simulink model "arducopter"  (R2021a)
settings: Solver=FixedStepAuto  StartTime=0.0  StopTime=simIn.param.timeEnd  FixedStep=simIn.param.dt  RelTol=1e-3
undefined symbols (not defined in the file or in its folder): DiscIntNeverNeededParam, sim, simIn
libraries: simulink x35, slident x4, vrlib x1
(part 3 of 9)

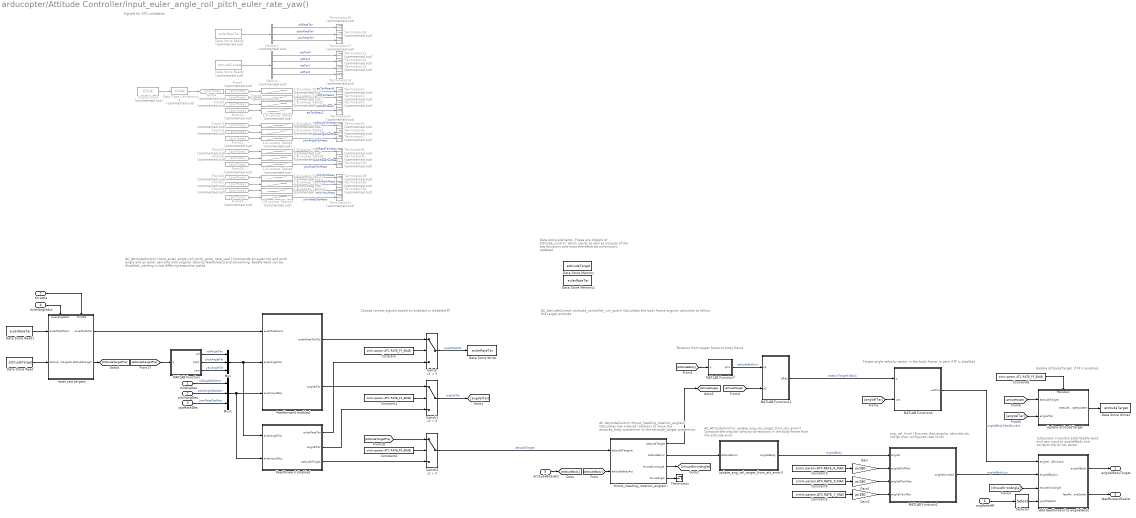
== system arducopter/Attitude Controller/input_euler_angle_roll_pitch_euler_rate_yaw() ==
  note: Signals for SITL validation
  note: Data store elements. These are objects of attitude_control, which inputs as well as outputs of the two functions and must therefore be continously updated
  note: Update attitudeTarget, if FF is enabled.
  note: Subsystem smoothly adds feedforward and yaw input to angVelBody and corrects the thrust vector
  note: Target angle velocity vector in the body frame. Is zero if FF is disabled
  note: Rotation from target frame to body frame
  note: Choose correct signals based on enabled or disabled FF
  note: AC_AttitudeControl::input_euler_angle_roll_pitch_euler_rate_yaw()
      | Commands an euler roll and pitch angle and an euler yaw arte with angular velocity feedforward and smoothing.
      | Feedforward can be disabled, yielding in two differing execution paths.
  note: AC_AttitudeControl::thrust_heading_rotation_angles()
      | Calculates two ordered rotations to move the attitude_body quaternion to the attitude_target quaternion.
  note: AC_AttitudeControl::update_ang_vel_target_from_att_error()
      | Compute the angular velocity corrections in the body frame from the attitude error.
  note: ang_vel_limit()
      | Ensures that angular velocites do not go over configured rate limits
  note: AC_AttitudeControl::attitude_controller_run_quat()
      | Calculates the body frame angular velocities to follow the target attitude
  rollAngDes : Inport
  pitchAngDes : Inport  Port=2
  yawRateDes : Inport  Port=3
  eulerAngleAct : Inport  Port=4
  attitudeBodyAct : Inport  Port=5
  angRatesBf : Inport  Port=6
  throttle : Inport  Port=7
  1-D Lookup Table : Lookup_n-D  Commented=on  NumberOfTableDimensions=1  BreakpointsForDimension1=simIn.signals.ATT.Time  Table=simIn.signals.ATT.attTarMeasW  InternalRulePriority=Speed  RndMeth=Simplest  InputSameDT=on
  1-D Lookup Table1 : Lookup_n-D  Commented=on  NumberOfTableDimensions=1  BreakpointsForDimension1=simIn.signals.ATT.Time  Table=simIn.signals.ATT.attTarMeasX  InternalRulePriority=Speed  RndMeth=Simplest  InputSameDT=on
  1-D Lookup Table10 : Lookup_n-D  Commented=on  NumberOfTableDimensions=1  BreakpointsForDimension1=simIn.signals.ATT.Time  Table=simIn.signals.ATT.CtrlRollIn  InternalRulePriority=Speed  RndMeth=Simplest  InputSameDT=on
  1-D Lookup Table11 : Lookup_n-D  Commented=on  NumberOfTableDimensions=1  BreakpointsForDimension1=simIn.signals.ATT.Time  Table=simIn.signals.ATT.CtrlPitchIn  InternalRulePriority=Speed  RndMeth=Simplest  InputSameDT=on
  1-D Lookup Table12 : Lookup_n-D  Commented=on  NumberOfTableDimensions=1  BreakpointsForDimension1=simIn.signals.ATT.Time  Table=simIn.signals.ATT.CtrlYawIn  InternalRulePriority=Speed  RndMeth=Simplest  InputSameDT=on
  1-D Lookup Table13 : Lookup_n-D  Commented=on  NumberOfTableDimensions=1  BreakpointsForDimension1=simIn.signals.ATT.Time  Table=simIn.signals.ATT.yawRateDesMeas  InternalRulePriority=Speed  RndMeth=Simplest  InputSameDT=on
  1-D Lookup Table2 : Lookup_n-D  Commented=on  NumberOfTableDimensions=1  BreakpointsForDimension1=simIn.signals.ATT.Time  Table=simIn.signals.ATT.attTarMeasY  InternalRulePriority=Speed  RndMeth=Simplest  InputSameDT=on
  1-D Lookup Table3 : Lookup_n-D  Commented=on  NumberOfTableDimensions=1  BreakpointsForDimension1=simIn.signals.ATT.Time  Table=simIn.signals.ATT.attTarMeasZ  InternalRulePriority=Speed  RndMeth=Simplest  InputSameDT=on
  1-D Lookup Table4 : Lookup_n-D  Commented=on  NumberOfTableDimensions=1  BreakpointsForDimension1=simIn.signals.ATT.Time  Table=simIn.signals.ATT.eulerAngTarMeasX  InternalRulePriority=Speed  RndMeth=Simplest  InputSameDT=on
  1-D Lookup Table5 : Lookup_n-D  Commented=on  NumberOfTableDimensions=1  BreakpointsForDimension1=simIn.signals.ATT.Time  Table=simIn.signals.ATT.eulerAngTarMeasY  InternalRulePriority=Speed  RndMeth=Simplest  InputSameDT=on
  1-D Lookup Table6 : Lookup_n-D  Commented=on  NumberOfTableDimensions=1  BreakpointsForDimension1=simIn.signals.ATT.Time  Table=simIn.signals.ATT.eulerAngTarMeasZ  InternalRulePriority=Speed  RndMeth=Simplest  InputSameDT=on
  1-D Lookup Table7 : Lookup_n-D  Commented=on  NumberOfTableDimensions=1  BreakpointsForDimension1=simIn.signals.ATT.Time  Table=simIn.signals.ATT.eulerRatTarMeasX  InternalRulePriority=Speed  RndMeth=Simplest  InputSameDT=on
  1-D Lookup Table8 : Lookup_n-D  Commented=on  NumberOfTableDimensions=1  BreakpointsForDimension1=simIn.signals.ATT.Time  Table=simIn.signals.ATT.eulerRatTarMeasY  InternalRulePriority=Speed  RndMeth=Simplest  InputSameDT=on
  1-D Lookup Table9 : Lookup_n-D  Commented=on  NumberOfTableDimensions=1  BreakpointsForDimension1=simIn.signals.ATT.Time  Table=simIn.signals.ATT.eulerRatTarMeasZ  InternalRulePriority=Speed  RndMeth=Simplest  InputSameDT=on
  Add feedforward to angVelBody : Subsystem
  Constant{,1..2,6} (4 alike) : Constant  Value=simIn.param.ATC.RATE_FF_ENAB
  Constant3 : Constant  Value=simIn.param.ATC.RATE_R_MAX
  Constant4 : Constant  Value=simIn.param.ATC.RATE_P_MAX
  Constant5 : Constant  Value=simIn.param.ATC.RATE_Y_MAX
  Data Store Memory : DataStoreMemory  DataStoreName=attitudeTarget  ReadBeforeWriteMsg=warning  WriteAfterWriteMsg=warning  WriteAfterReadMsg=warning  InitialValue=simIn.init.ATT.attitudeTarget  ShowAdditionalParam=off  OutDataTypeStr=single
  Data Store Memory1 : DataStoreMemory  DataStoreName=eulerRateTar  ReadBeforeWriteMsg=warning  WriteAfterWriteMsg=warning  WriteAfterReadMsg=warning  InitialValue=simIn.init.ATT.eulerRateTar  ShowAdditionalParam=off  OutDataTypeStr=single
  Data Store Read : DataStoreRead  DataStoreName=attitudeTarget  IndexOptions=Index vector (dialog)  Indices=1  OutputSizes=1
  Data Store Read1 : DataStoreRead  DataStoreName=eulerRateTar  IndexOptions=Index vector (dialog)  Indices=1  OutputSizes=1
  Data Store Read3 : DataStoreRead  Commented=on  DataStoreName=attitudeTarget  IndexOptions=Index vector (dialog)  Indices=1  OutputSizes=1
  Data Store Read4 : DataStoreRead  Commented=on  DataStoreName=eulerRateTar  IndexOptions=Index vector (dialog)  Indices=1  OutputSizes=1
  Data Store Write : DataStoreWrite  DataStoreName=eulerRateTar  IndexOptions=Index vector (dialog)  Indices=1  OutputSizes=1
  Data Store Write1 : DataStoreWrite  DataStoreName=attitudeTarget  IndexOptions=Index vector (dialog)  Indices=1  OutputSizes=1
  Data Type Conversion4 : DataTypeConversion  Commented=on  OutDataTypeStr=single
  Demux : Demux  Commented=on
  Demux1 : Demux  Commented=on  Outputs=3
  Digital Clock : DigitalClock  Commented=on  SampleTime=sim.param.dt
  Feedforward disabled : Subsystem
  Feedforward enabled : Subsystem
  From{7..16,19..22} (14 alike) : From  Commented=on  GotoTag=simTime
  Gain : Gain  Gain=pi/180
  Gain1 : Gain  Gain=pi/180
  Gain2 : Gain  Gain=pi/180
  Goto4 : Goto  Commented=on  GotoTag=simTime
  MATLAB Function : MATLAB Function  TreatAsAtomicUnit=on
  MATLAB Function11 : MATLAB Function  TreatAsAtomicUnit=on
  MATLAB Function2 : MATLAB Function  TreatAsAtomicUnit=on
  MATLAB Function4 : MATLAB Function  TreatAsAtomicUnit=on
  MATLAB Function7 : MATLAB Function  TreatAsAtomicUnit=on
  Mux : Mux  Inputs=3
  Mux1 : Mux  Inputs=3
  Selector : Selector  InputPortWidth=3  IndexOptions=Index vector (dialog)  Indices=[3]  OutputSizes=1
  Switch : Switch  Criteria=u2 > Threshold
  Switch1 : Switch  Criteria=u2 > Threshold
  Switch2 : Switch  Criteria=u2 > Threshold
  Terminator : Terminator
  Terminator{1..21} (21 alike) : Terminator  Commented=on
  Update attitudeTarget : Subsystem
      settings: PortSchema="{\"entries\":[{\"content\":{\"sides\":[{\"content\":{\"connectorIds\":[\"In1\",\"In2\"]},\"type\":\"ConnectorPlacement.EquallySpacedRectSide\",\"uuid\":\"677f2474-a933-4351-a18c-d191f7c74006\"},{\"content\":{\"connectorIds\":[\"Out1\"],\"side\":\"RIGHT\"},\"type\":\"ConnectorPlacement.EquallySpacedRectSide\",\"uuid\":\"e9b9097f-3644-4a9a-8149-04c97bd90a0c\"},{\"content\":{\"connectorIds\":[\"In3\"],\"side\":\"TOP\"},\"type\":\"ConnectorPlacement.EquallySpacedRectSide\",\"uuid\":\"2b4d5a13-4fc6-40d8-be4c-f1f4571d6c96\"}]},\"type\":\"ConnectorPlacement.EquallySpacedConnector\",\"uuid\":\"62980eaf-3b78-41ff-aa7a-c4a8a9508ced\"}],\"packageUris\":[\"http://schema.mathworks.com/mf0/Connector/R2020b\"],\"version\":\"1.0\"}"
  reset yaw targets : Subsystem
      settings: PortSchema="{\"entries\":[{\"content\":{\"sides\":[{\"content\":{\"connectorIds\":[\"In1\",\"In2\"]},\"type\":\"ConnectorPlacement.EquallySpacedRectSide\",\"uuid\":\"29284c76-4388-4ab2-b640-2aa249641a5e\"},{\"content\":{\"connectorIds\":[\"Out1\",\"Out2\"],\"side\":\"RIGHT\"},\"type\":\"ConnectorPlacement.EquallySpacedRectSide\",\"uuid\":\"b3687b33-33ad-4cf1-ba70-eea9295fb5e4\"},{\"content\":{\"connectorIds\":[\"In3\",\"In4\"],\"side\":\"TOP\"},\"type\":\"ConnectorPlacement.EquallySpacedRectSide\",\"uuid\":\"b547cb73-472d-403b-8f7c-c78a9fbe5228\"}]},\"type\":\"ConnectorPlacement.EquallySpacedConnector\",\"uuid\":\"31dffed6-fd3b-4288-90b3-a2b7b520dc2f\"}],\"packageUris\":[\"http://schema.mathworks.com/mf0/Connector/R2020b\"],\"version\":\"1.0\"}"
  thrust_heading_rotation_angles() : Subsystem
  update_ang_vel_target_from_att_error() : Subsystem
  angVelBodyTarget : Outport
  feedforwardScaler : Outport  Port=2
  wires:
  MATLAB Function/3(yaw) -> Mux/3  "yawAngleTar"
  MATLAB Function/2(pitch) -> Mux/2  "pitchAngleTar"
  MATLAB Function/1(roll) -> Mux/1  "rollAngleTar"
  Mux/1 -> Feedforward disabled/1(eulerAngleTar), Feedforward enabled/2(eulerAngleTar)
  rollAngDes/1 -> Mux1/1  "rollAngleDesNew"
  pitchAngDes/1 -> Mux1/2  "pitchAngleDesNew"
  yawRateDes/1 -> Mux1/3  "yawRateDesNew"
  Mux1/1 -> Feedforward enabled/3(eulerInputDes), Feedforward disabled/2(eulerInputDes)
  Data Store Read1/1 -> reset yaw targets/1(eulerRateTarIn)
  Feedforward enabled/1(eulerRateTarOut) -> Switch/1
  Feedforward disabled/1(eulerRateTar) -> Switch/3
  Feedforward enabled/2(angVelTar) -> Switch1/1
  Constant/1 -> Switch/2
  Feedforward disabled/2(angVelTar) -> Switch1/3
  Switch/1 -> Data Store Write/1  "eulerRateTar"
  Switch1/1 -> [angVelTar]  "angVelTar"
  Constant1/1 -> Switch1/2
  Constant2/1 -> Switch2/2
  [attitudeTargetPre] -> Switch2/1
  Feedforward disabled/3(attitudeTarget) -> Switch2/3
  Switch2/1 -> thrust_heading_rotation_angles()/1(attitudeTargetIn)  "attitudeTarget"
  [attitudeBody] -> thrust_heading_rotation_angles()/2(attitudeBodyAct)
  thrust_heading_rotation_angles()/4(thrustAngle) -> Terminator/1
  thrust_heading_rotation_angles()/2(attitudeError) -> update_ang_vel_target_from_att_error()/1(attitudeError)
  Constant4/1 -> Gain1/1
  Constant3/1 -> Gain/1
  Gain2/1 -> MATLAB Function2/4(angVelYawMax)
  Gain1/1 -> MATLAB Function2/3(angVelPitchMax)
  Constant5/1 -> Gain2/1
  Gain/1 -> MATLAB Function2/2(angVelRollMax)
  update_ang_vel_target_from_att_error()/1(angVelBody) -> MATLAB Function2/1(angVel)  "angVelBody"
  attitudeBodyAct/1 -> [attitudeBody]
  thrust_heading_rotation_angles()/1(attitudeTarget) -> [attitudeTarget]
  [attitudeBody] -> MATLAB Function7/1(q)
  MATLAB Function7/1(qInv) -> MATLAB Function11/1(q1)  "attitudeBodyInv"
  MATLAB Function11/1(qRes) -> MATLAB Function4/1(q)  "rotationTargetToBody"
  [angVelTar] -> MATLAB Function4/2(vec)
  MATLAB Function4/1(vecRot) -> Add feedforward to angVelBody/1(angVelBodyFeedforward)  "angVelBodyFeedforward"
  thrust_heading_rotation_angles()/3(thrustErrorAngle) -> [thrustErrorAngle]
  MATLAB Function2/1(angVelLimited) -> Add feedforward to angVelBody/2(angVelBodyIn)  "angVelBodyLim"
  [thrustErrorAngle] -> Add feedforward to angVelBody/3(thurstErrorAngle)
  angRatesBf/1 -> Selector/1
  Selector/1 -> Add feedforward to angVelBody/4(yawRateAct)
  [attitudeTarget] -> MATLAB Function11/2(q2)
  [angVelTar] -> Update attitudeTarget/2(angVelTar)
  Add feedforward to angVelBody/1(angVelBody) -> angVelBodyTarget/1
  [attitudeTarget] -> Update attitudeTarget/1(attitudeTarget)
  Update attitudeTarget/1(attitudeTargetUpdate) -> Data Store Write1/1
  Constant6/1 -> Update attitudeTarget/3(ffEnabled)
  Add feedforward to angVelBody/2(feedforwardScaler) -> feedforwardScaler/1
  Data Type Conversion4/1 -> Goto4/1
  Digital Clock/1 -> Data Type Conversion4/1
  From7/1 -> 1-D Lookup Table/1
  From8/1 -> 1-D Lookup Table1/1
  From9/1 -> 1-D Lookup Table2/1
  From10/1 -> 1-D Lookup Table3/1
  From11/1 -> 1-D Lookup Table6/1
  From13/1 -> 1-D Lookup Table5/1
  From12/1 -> 1-D Lookup Table4/1
  From15/1 -> 1-D Lookup Table7/1
  From16/1 -> 1-D Lookup Table8/1
  From14/1 -> 1-D Lookup Table9/1
  1-D Lookup Table/1 -> Terminator1/1  "attTarMeasW"
  1-D Lookup Table1/1 -> Terminator2/1  "attTarMeasX"
  1-D Lookup Table2/1 -> Terminator3/1  "attTarMeasY"
  1-D Lookup Table3/1 -> Terminator4/1  "attTarMeasZ"
  1-D Lookup Table6/1 -> Terminator7/1  "yawAngleTarMeas"
  1-D Lookup Table5/1 -> Terminator6/1  "pitchAngleTarMeas"
  1-D Lookup Table4/1 -> Terminator5/1  "rollAngleTarMeas"
  1-D Lookup Table7/1 -> Terminator8/1  "rollRateTarMeas"
  1-D Lookup Table8/1 -> Terminator9/1  "pitchRateTarMeas"
  1-D Lookup Table9/1 -> Terminator10/1  "yawRateTarMeas"
  Data Store Read3/1 -> Demux/1
  Demux/4 -> Terminator14/1  "attTarZ"
  Demux/3 -> Terminator13/1  "attTarY"
  Demux/2 -> Terminator12/1  "attTarX"
  Demux/1 -> Terminator11/1  "attTarW"
  Data Store Read4/1 -> Demux1/1
  Demux1/1 -> Terminator15/1  "rollRateTar"
  Demux1/2 -> Terminator16/1  "pitchRateTar"
  Demux1/3 -> Terminator17/1  "yawRateTar"
  Data Store Read/1 -> reset yaw targets/2(attitudeTargetIn)
  reset yaw targets/1(eulerRateTar) -> Feedforward enabled/1(eulerRateTarIn)
  eulerAngleAct/1 -> reset yaw targets/3(eulerAngleAct)
  [attitudeTargetPre] -> MATLAB Function/1(q)
  reset yaw targets/2(attitudeTarget) -> [attitudeTargetPre]
  throttle/1 -> reset yaw targets/4(throttle)
  From19/1 -> 1-D Lookup Table12/1
  From21/1 -> 1-D Lookup Table11/1
  From20/1 -> 1-D Lookup Table10/1
  From22/1 -> 1-D Lookup Table13/1
  1-D Lookup Table10/1 -> Terminator19/1  "ctrlInRollMeas"
  1-D Lookup Table11/1 -> Terminator20/1  "ctrlInPitchMeas"
  1-D Lookup Table12/1 -> Terminator18/1  "ctrlInYawMeas"
  1-D Lookup Table13/1 -> Terminator21/1  "yawRateDesMeas"

== system arducopter/Lowpass2p/Lowpass Pitch ==
  u : Inport
  sampleFreq : Inport  Port=2
  cutoffFreq : Inport  Port=3
  Data Store Memory1 : DataStoreMemory  DataStoreName=delElem2  ReadBeforeWriteMsg=warning  WriteAfterWriteMsg=warning  WriteAfterReadMsg=warning  ShowAdditionalParam=off  OutDataTypeStr=single
  Data Store Memory10 : DataStoreMemory  DataStoreName=delElem1  ReadBeforeWriteMsg=warning  WriteAfterWriteMsg=warning  WriteAfterReadMsg=warning  ShowAdditionalParam=off  OutDataTypeStr=single
  Lowpass2p : MATLAB Function  TreatAsAtomicUnit=on
  y : Outport
  wires:
  u/1 -> Lowpass2p/1(u)
  cutoffFreq/1 -> Lowpass2p/3(cutoffFreq)
  sampleFreq/1 -> Lowpass2p/2(sampleFreq)
  Lowpass2p/1(y) -> y/1

== system arducopter/Lowpass2p/Lowpass Roll ==
  u : Inport
  sampleFreq : Inport  Port=2
  cutoffFreq : Inport  Port=3
  Data Store Memory1 : DataStoreMemory  DataStoreName=delElem2  ReadBeforeWriteMsg=warning  WriteAfterWriteMsg=warning  WriteAfterReadMsg=warning  ShowAdditionalParam=off  OutDataTypeStr=single
  Data Store Memory10 : DataStoreMemory  DataStoreName=delElem1  ReadBeforeWriteMsg=warning  WriteAfterWriteMsg=warning  WriteAfterReadMsg=warning  ShowAdditionalParam=off  OutDataTypeStr=single
  Lowpass2p : MATLAB Function  TreatAsAtomicUnit=on
  y : Outport
  wires:
  Lowpass2p/1(y) -> y/1
  sampleFreq/1 -> Lowpass2p/2(sampleFreq)
  cutoffFreq/1 -> Lowpass2p/3(cutoffFreq)
  u/1 -> Lowpass2p/1(u)

== system arducopter/Lowpass2p/Lowpass Yaw ==
  u : Inport
  sampleFreq : Inport  Port=2
  cutoffFreq : Inport  Port=3
  Data Store Memory1 : DataStoreMemory  DataStoreName=delElem2  ReadBeforeWriteMsg=warning  WriteAfterWriteMsg=warning  WriteAfterReadMsg=warning  ShowAdditionalParam=off  OutDataTypeStr=single
  Data Store Memory10 : DataStoreMemory  DataStoreName=delElem1  ReadBeforeWriteMsg=warning  WriteAfterWriteMsg=warning  WriteAfterReadMsg=warning  ShowAdditionalParam=off  OutDataTypeStr=single
  Lowpass2p : MATLAB Function  TreatAsAtomicUnit=on
  y : Outport
  wires:
  u/1 -> Lowpass2p/1(u)
  cutoffFreq/1 -> Lowpass2p/3(cutoffFreq)
  sampleFreq/1 -> Lowpass2p/2(sampleFreq)
  Lowpass2p/1(y) -> y/1

== system arducopter/Position Controller/P Position z ==
  note: AC_PosControl::update_z_controller() - Position controller
  note: Feed-Forward component
      | update_z_controller()
  note: AC_P_1D::update_all()
      | These two Matlab functions represent the update_all() function of the AC_P_1D class. The function basically consists of two parts, the error
      | calculation with limiting (implemented by calc_err) and the square root controller (implemented by sqrt_controller).
  note: Testrun inputs
  note: Parameter
  note: AC_PosControl::set_correction_speed_accel_z()
  posTar : Inport
  posAct : Inport  Port=2
  velDes : Inport  Port=3
  Calculate error : MATLAB Function  TreatAsAtomicUnit=on
  Constant : Constant  Value=0  OutDataTypeStr=single
  Data Type Conversion : DataTypeConversion  OutDataTypeStr=single
  IC1 : InitialCondition  Value=simIn.init.PIDA.posTar
  Product : Product
  Scale Factor Z : Subsystem
  Set vertical speed & acceleration limit : Subsystem
  Square Root Controller : MATLAB Function  TreatAsAtomicUnit=on
  Sum : Sum  Inputs=++|
  dt : Constant  Value=simIn.param.dt
  ekf_type : Constant  Value=simIn.param.EKF_TYPE
  kp_pos : Constant  Value=simIn.param.PSCD.P_POS
  speedDnMax : Constant  Value=simIn.param.PSCD.VEL_MAX_DN
  speedUpMax : Constant  Value=simIn.param.PSCD.VEL_MAX_UP
  zAccMax : Constant  Value=simIn.param.PSCD.ACC_MAX_Z
  velTar : Outport
  posTarUpd : Outport  Port=2
  posErr : Outport  Port=3
  wires:
  speedDnMax/1 -> [dnSpeedMax]
  posAct/1 -> Calculate error/2(act)
  posTar/1 -> IC1/1
  speedUpMax/1 -> [upSpeedMax]
  zAccMax/1 -> [zAccMax]
  kp_pos/1 -> [kpPos]
  [errMin] -> Calculate error/3(err_min)
  [errMax] -> Calculate error/4(err_max)
  [dnSpeedMax] -> Set vertical speed & acceleration limit/1(outMin)
  [upSpeedMax] -> Set vertical speed & acceleration limit/2(outMax)
  [zAccMax] -> Set vertical speed & acceleration limit/3(DoutMax)
  Constant/1 -> Set vertical speed & acceleration limit/4(D2OutMax)
  Set vertical speed & acceleration limit/1(errMin) -> [errMin]
  Set vertical speed & acceleration limit/2(errMax) -> [errMax]
  [error] -> Square Root Controller/1(err)
  Set vertical speed & acceleration limit/3(D1max) -> [D1max]
  [D1max] -> Square Root Controller/3(second_ord_lim)
  [kpPos] -> Square Root Controller/2(p)
  dt/1 -> Data Type Conversion/1
  [dt] -> Square Root Controller/4(dt)
  ekf_type/1 -> [ekfType]
  [ekfType] -> Scale Factor Z/1(ekfType)
  Square Root Controller/1(correction_rate) -> Product/2
  Scale Factor Z/1(scale_z) -> Product/1
  Calculate error/1(tar_new) -> posTarUpd/1
  Product/1 -> Sum/2
  velDes/1 -> Sum/1
  Sum/1 -> velTar/1
  Data Type Conversion/1 -> [dt]
  IC1/1 -> Calculate error/1(tar)
  Calculate error/2(err) -> [error]
  [error] -> posErr/1
  [kpPos] -> Set vertical speed & acceleration limit/5(kp)

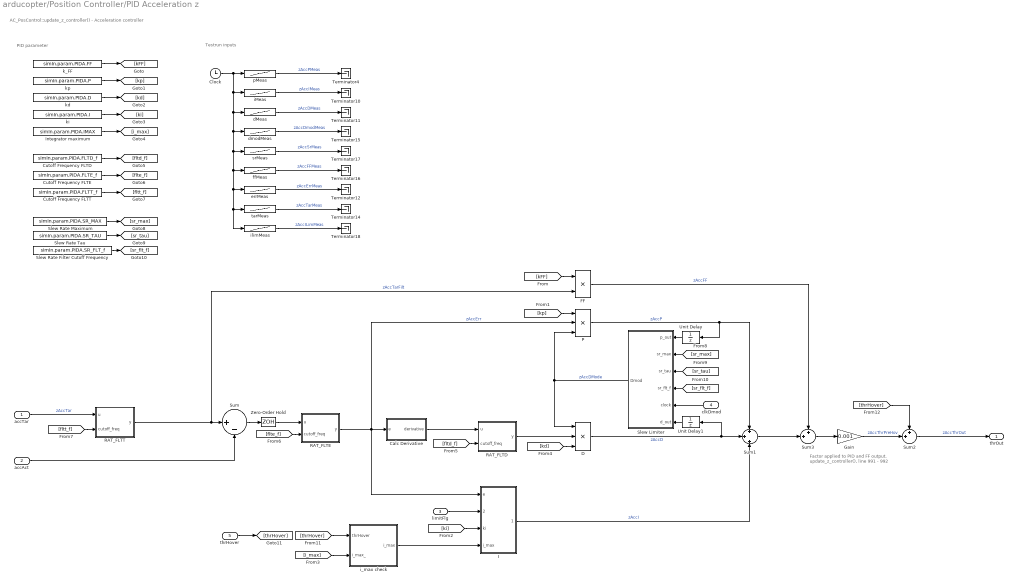
== system arducopter/Position Controller/PID Acceleration z ==
  note: Factor applied to PID and FF output.
      | update_z_controller(), line 991 - 992
  note: AC_PosControl::update_z_controller() - Acceleration controller
  note: PID parameter
  note: Testrun inputs
  accTar : Inport
  accAct : Inport  Port=2
  limitFlg : Inport  Port=3
  clkDmod : Inport  Port=4
  thrHover : Inport  Port=5
  Calc Derivative : Subsystem
  Clock : Clock
  Cutoff Frequency FLTD : Constant  Value=simIn.param.PIDA.FLTD_f
  Cutoff Frequency FLTE : Constant  Value=simIn.param.PIDA.FLTE_f
  Cutoff Frequency FLTT : Constant  Value=simIn.param.PIDA.FLTT_f
  D : Product  Inputs=3
  FF : Product
  Gain : Gain  Gain=0.001
  I : Subsystem
  Integrator maximum : Constant  Value=simIn.param.PIDA.IMAX
  P : Product  Inputs=3
  RAT_FLTD : Subsystem  TreatAsAtomicUnit=on  SystemSampleTime=simIn.param.dt
  RAT_FLTE : Subsystem  TreatAsAtomicUnit=on  SystemSampleTime=simIn.param.dt
  RAT_FLTT : Subsystem  TreatAsAtomicUnit=on  SystemSampleTime=simIn.param.dt
  Slew Limiter : Subsystem
  Slew Rate Filter Cutoff Frequency : Constant  Value=simIn.param.PIDA.SR_FLT_f
  Slew Rate Maximum : Constant  Value=simIn.param.PIDA.SR_MAX
  Slew Rate Tau : Constant  Value=simIn.param.PIDA.SR_TAU
  Sum : Sum  Inputs=|+-
  Sum1 : Sum  Inputs=+|+|+
  Sum2 : Sum  Inputs=++|  OutDataTypeStr=single
  Sum3 : Sum  Inputs=++|  OutDataTypeStr=single
  Terminator{4,10..12,14..18} (9 alike) : Terminator
  Unit Delay : UnitDelay  InitialCondition=simIn.init.PIDA.P  SampleTime=-1  HasFrameUpgradeWarning=on
  Unit Delay1 : UnitDelay  InitialCondition=simIn.init.PIDA.D  SampleTime=-1  HasFrameUpgradeWarning=on
  Zero-Order Hold : ZeroOrderHold  SampleTime=-1
  dMeas : Lookup_n-D  NumberOfTableDimensions=1  BreakpointsForDimension1=simIn.signals.PIDR.Time  Table=simIn.signals.PIDR.D  InternalRulePriority=Speed  RndMeth=Simplest  InputSameDT=on
  dmodMeas : Lookup_n-D  NumberOfTableDimensions=1  BreakpointsForDimension1=simIn.signals.PIDA.Time  Table=simIn.signals.PIDA.DMod  InternalRulePriority=Speed  RndMeth=Simplest  InputSameDT=on
  errMeas : Lookup_n-D  NumberOfTableDimensions=1  BreakpointsForDimension1=simIn.signals.PIDA.Time  Table=simIn.signals.PIDA.Err  InternalRulePriority=Speed  RndMeth=Simplest  InputSameDT=on
  ffMeas : Lookup_n-D  NumberOfTableDimensions=1  BreakpointsForDimension1=simIn.signals.PIDA.Time  Table=simIn.signals.PIDA.FF  InternalRulePriority=Speed  RndMeth=Simplest  InputSameDT=on
  iMeas : Lookup_n-D  NumberOfTableDimensions=1  BreakpointsForDimension1=simIn.signals.PIDA.Time  Table=simIn.signals.PIDA.I  InternalRulePriority=Speed  RndMeth=Simplest  InputSameDT=on
  i_max check : Subsystem
  ilimMeas : Lookup_n-D  NumberOfTableDimensions=1  BreakpointsForDimension1=simIn.signals.PIDA.Time  Table=simIn.signals.PIDA.ILimit  InternalRulePriority=Speed  RndMeth=Simplest  InputSameDT=on
  k_FF : Constant  Value=simIn.param.PIDA.FF
  kd : Constant  Value=simIn.param.PIDA.D
  ki : Constant  Value=simIn.param.PIDA.I
  kp : Constant  Value=simIn.param.PIDA.P
  pMeas : Lookup_n-D  NumberOfTableDimensions=1  BreakpointsForDimension1=simIn.signals.PIDA.Time  Table=simIn.signals.PIDA.P  InternalRulePriority=Speed  RndMeth=Simplest  InputSameDT=on
  srMeas : Lookup_n-D  NumberOfTableDimensions=1  BreakpointsForDimension1=simIn.signals.PIDA.Time  Table=simIn.signals.PIDA.SRate  InternalRulePriority=Speed  RndMeth=Simplest  InputSameDT=on
  tarMeas : Lookup_n-D  NumberOfTableDimensions=1  BreakpointsForDimension1=simIn.signals.PSCD.Time  Table=simIn.signals.PSCD.zAccTar  InternalRulePriority=Speed  RndMeth=Simplest  InputSameDT=on
  thrOut : Outport
  wires:
  RAT_FLTD/1(y) -> D/2
  Sum1/1 -> Sum3/2
  limitFlg/1 -> I/2(limitFlg)
  P/1 -> Unit Delay/1, Sum1/1  "zAccP"
  Calc Derivative/1(derivative) -> RAT_FLTD/1(u)
  Sum/1 -> Zero-Order Hold/1
  D/1 -> Unit Delay1/1, Sum1/2  "zAccD"
  I/1(integrator) -> Sum1/3  "zAccI"
  FF/1 -> Sum3/1  "zAccFF"
  Sum3/1 -> Gain/1
  RAT_FLTT/1(y) -> FF/2, Sum/1  "zAccTarFilt"
  Zero-Order Hold/1 -> RAT_FLTE/1(u)
  k_FF/1 -> [kFF]
  kp/1 -> [kp]
  kd/1 -> [kd]
  ki/1 -> [ki]
  Integrator maximum/1 -> [i_max]
  Cutoff Frequency FLTD/1 -> [fltd_f]
  Cutoff Frequency FLTE/1 -> [flte_f]
  Cutoff Frequency FLTT/1 -> [fltt_f]
  [kFF] -> FF/1
  [kp] -> P/1
  [ki] -> I/3(ki)
  [kd] -> D/3
  [fltd_f] -> RAT_FLTD/2(cutoff_freq)
  [flte_f] -> RAT_FLTE/2(cutoff_freq)
  [fltt_f] -> RAT_FLTT/2(cutoff_freq)
  RAT_FLTE/1(y) -> P/2, Calc Derivative/1(e), I/1(e)  "zAccErr"
  Slew Rate Filter Cutoff Frequency/1 -> [sr_flt_f]
  Slew Rate Maximum/1 -> [sr_max]
  Slew Rate Tau/1 -> [sr_tau]
  Slew Limiter/1(Dmod) -> D/1, P/3  "zAccDMode"
  Unit Delay/1 -> Slew Limiter/1(p_out)
  Unit Delay1/1 -> Slew Limiter/6(d_out)
  [sr_max] -> Slew Limiter/2(sr_max)
  [sr_tau] -> Slew Limiter/3(sr_tau)
  [sr_flt_f] -> Slew Limiter/4(sr_flt_f)
  clkDmod/1 -> Slew Limiter/5(clock)
  [thrHover] -> i_max check/1(thrHover)
  [i_max] -> i_max check/2(i_max_)
  i_max check/1(i_max) -> I/4(i_max)
  Sum2/1 -> thrOut/1  "zAccThrOut"
  thrHover/1 -> [thrHover]
  Gain/1 -> Sum2/2  "zAccThrPreHov"
  [thrHover] -> Sum2/1
  Clock/1 -> ilimMeas/1, tarMeas/1, errMeas/1, ffMeas/1, srMeas/1, dmodMeas/1, dMeas/1, iMeas/1, pMeas/1
  dmodMeas/1 -> Terminator15/1  "zAccDmodMeas"
  ilimMeas/1 -> Terminator18/1  "zAccILimMeas"
  srMeas/1 -> Terminator17/1  "zAccSrMeas"
  iMeas/1 -> Terminator10/1  "zAccIMeas"
  ffMeas/1 -> Terminator16/1  "zAccFFMeas"
  pMeas/1 -> Terminator4/1  "zAccPMeas"
  errMeas/1 -> Terminator12/1  "zAccErrMeas"
  tarMeas/1 -> Terminator14/1  "zAccTarMeas"
  dMeas/1 -> Terminator11/1  "zAccDMeas"
  accAct/1 -> Sum/2
  accTar/1 -> RAT_FLTT/1(u)  "zAccTar"

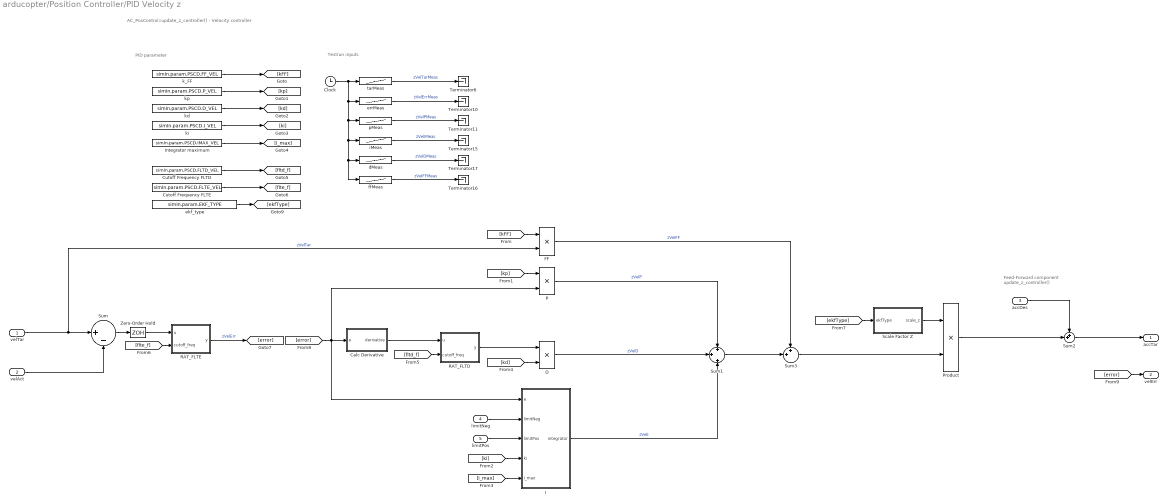
== system arducopter/Position Controller/PID Velocity z ==
  note: PID parameter
  note: Testrun inputs
  note: Feed-Forward component
      | update_z_controller()
  note: AC_PosControl::update_z_controller() - Velocity controller
  velTar : Inport
  velAct : Inport  Port=2
  accDes : Inport  Port=3
  limitNeg : Inport  Port=4
  limitPos : Inport  Port=5
  Calc Derivative : Subsystem
  Clock : Clock
  Cutoff Frequency FLTD : Constant  Value=simIn.param.PSCD.FLTD_VEL
  Cutoff Frequency FLTE : Constant  Value=simIn.param.PSCD.FLTE_VEL
  D : Product
  FF : Product
  I : Subsystem
  Integrator maximum : Constant  Value=simIn.param.PSCD.IMAX_VEL
  P : Product
  Product : Product
  RAT_FLTD : Subsystem  TreatAsAtomicUnit=on  SystemSampleTime=simIn.param.dt
  RAT_FLTE : Subsystem  TreatAsAtomicUnit=on  SystemSampleTime=simIn.param.dt
  Scale Factor Z : Subsystem
  Sum : Sum  Inputs=|+-
  Sum1 : Sum  Inputs=+|+|+
  Sum2 : Sum  Inputs=++|
  Sum3 : Sum  Inputs=++|  OutDataTypeStr=single
  Terminator{6,10..11,15..17} (6 alike) : Terminator
  Zero-Order Hold : ZeroOrderHold  SampleTime=-1
  dMeas : Lookup_n-D  NumberOfTableDimensions=1  BreakpointsForDimension1=simIn.signals.PCVZ.Time  Table=simIn.signals.PCVZ.D  InternalRulePriority=Speed  RndMeth=Simplest  InputSameDT=on
  ekf_type : Constant  Value=simIn.param.EKF_TYPE
  errMeas : Lookup_n-D  NumberOfTableDimensions=1  BreakpointsForDimension1=simIn.signals.PCVZ.Time  Table=simIn.signals.PCVZ.Err  InternalRulePriority=Speed  RndMeth=Simplest  InputSameDT=on
  ffMeas : Lookup_n-D  NumberOfTableDimensions=1  BreakpointsForDimension1=simIn.signals.PCVZ.Time  Table=simIn.signals.PCVZ.FF  InternalRulePriority=Speed  RndMeth=Simplest  InputSameDT=on
  iMeas : Lookup_n-D  NumberOfTableDimensions=1  BreakpointsForDimension1=simIn.signals.PCVZ.Time  Table=simIn.signals.PCVZ.I  InternalRulePriority=Speed  RndMeth=Simplest  InputSameDT=on
  k_FF : Constant  Value=simIn.param.PSCD.FF_VEL
  kd : Constant  Value=simIn.param.PSCD.D_VEL
  ki : Constant  Value=simIn.param.PSCD.I_VEL
  kp : Constant  Value=simIn.param.PSCD.P_VEL
  pMeas : Lookup_n-D  NumberOfTableDimensions=1  BreakpointsForDimension1=simIn.signals.PCVZ.Time  Table=simIn.signals.PCVZ.P  InternalRulePriority=Speed  RndMeth=Simplest  InputSameDT=on
  tarMeas : Lookup_n-D  NumberOfTableDimensions=1  BreakpointsForDimension1=simIn.signals.PSCD.Time  Table=simIn.signals.PSCD.zVelTar  InternalRulePriority=Speed  RndMeth=Simplest  InputSameDT=on
  accTar : Outport
  velErr : Outport  Port=2
  wires:
  RAT_FLTD/1(y) -> D/1
  Sum1/1 -> Sum3/2
  [error] -> I/1(e), P/2, Calc Derivative/1(e)
  limitNeg/1 -> I/2(limitNeg)
  P/1 -> Sum1/1  "zVelP"
  Calc Derivative/1(derivative) -> RAT_FLTD/1(u)
  Sum/1 -> Zero-Order Hold/1
  D/1 -> Sum1/2  "zVelD"
  I/1(integrator) -> Sum1/3  "zVelI"
  FF/1 -> Sum3/1  "zVelFF"
  velAct/1 -> Sum/2
  Zero-Order Hold/1 -> RAT_FLTE/1(u)
  k_FF/1 -> [kFF]
  kp/1 -> [kp]
  kd/1 -> [kd]
  ki/1 -> [ki]
  Integrator maximum/1 -> [i_max]
  Cutoff Frequency FLTD/1 -> [fltd_f]
  Cutoff Frequency FLTE/1 -> [flte_f]
  [kFF] -> FF/1
  [kp] -> P/1
  [ki] -> I/4(ki)
  [i_max] -> I/5(i_max)
  [kd] -> D/2
  [fltd_f] -> RAT_FLTD/2(cutoff_freq)
  [flte_f] -> RAT_FLTE/2(cutoff_freq)
  velTar/1 -> FF/2, Sum/1  "zVelTar"
  limitPos/1 -> I/3(limitPos)
  Sum3/1 -> Product/2
  [ekfType] -> Scale Factor Z/1(ekfType)
  Scale Factor Z/1(scale_z) -> Product/1
  accDes/1 -> Sum2/1
  Sum2/1 -> accTar/1
  Product/1 -> Sum2/2
  ekf_type/1 -> [ekfType]
  RAT_FLTE/1(y) -> [error]  "zVelErr"
  [error] -> velErr/1
  Clock/1 -> ffMeas/1, dMeas/1, iMeas/1, pMeas/1, errMeas/1, tarMeas/1
  tarMeas/1 -> Terminator6/1  "zVelTarMeas"
  pMeas/1 -> Terminator11/1  "zVelPMeas"
  ffMeas/1 -> Terminator16/1  "zVelFFMeas"
  dMeas/1 -> Terminator17/1  "zVelDMeas"
  iMeas/1 -> Terminator15/1  "zVelIMeas"
  errMeas/1 -> Terminator10/1  "zVelErrMeas"

== system arducopter/Position Controller/calc des climb rate ==
  note: Constrain target_climb_rate
  note: Calculation of desired climb rate from throttle control input.
      | Based on ModeAltHold::run(), where Copter::get_pilot_desired_climb_rate() is called from
  ctrlIn : Inport
  Constant1 : Constant  Value=simIn.param.PSCD.VEL_MAX_DN
  Constant18 : Constant  Value=simIn.param.PSCD.THR_DZ
  Constant19 : Constant  Value=simIn.param.RCIN.MIN_THR
  Constant2 : Constant  Value=simIn.param.PSCD.VEL_MAX_UP
  Constant20 : Constant  Value=simIn.param.RCIN.MAX_THR
  Constant21 : Constant  Value=simIn.param.RCIN.REVERSED_THR
  Constant22 : Constant  Value=1000
  Constant3 : Constant  Value=simIn.param.RCIN.DZ_THR
  MATLAB Function : MATLAB Function  TreatAsAtomicUnit=on
  constrain climb rate : Subsystem
  climbRate : Outport
  wires:
  ctrlIn/1 -> MATLAB Function/1(ctrlIn)
  MATLAB Function/1(climbRateDes) -> constrain climb rate/1(in)
  Constant18/1 -> MATLAB Function/2(deadZoneThr)
  Constant19/1 -> MATLAB Function/4(radioMin)
  Constant20/1 -> MATLAB Function/5(radioMax)
  Constant21/1 -> MATLAB Function/6(reversed)
  Constant22/1 -> MATLAB Function/7(highIn)
  Constant1/1 -> MATLAB Function/8(maxSpeedDn)
  Constant2/1 -> MATLAB Function/9(maxSpeedUp)
  constrain climb rate/1(out) -> climbRate/1
  Constant3/1 -> MATLAB Function/3(deadZoneRC)

== system arducopter/Position Controller/get_pilot_speed_dn() ==
  upMax : Inport
  MATLAB Function : MATLAB Function  TreatAsAtomicUnit=on
  dnSpeedMax : Constant  Value=simIn.param.PSCD.VEL_MAX_DN
  dnMax : Outport
  wires:
  dnSpeedMax/1 -> MATLAB Function/1(dnMaxIn)
  upMax/1 -> MATLAB Function/2(upMax)
  MATLAB Function/1(dnMax) -> dnMax/1

== system arducopter/Position Controller/input handler ==
  inSim : Inport
  inMeas : Inport  Port=2
  Constant : Constant  Value=simIn.param.mdlVal
  Switch : Switch  Criteria=u2 > Threshold
  inAct : Outport
  wires:
  inSim/1 -> Switch/1
  inMeas/1 -> Switch/3
  Switch/1 -> inAct/1
  Constant/1 -> Switch/2

== system arducopter/Position Controller/set z component of limit vec ==
  note: Set vertical component of limit vector based on throttle limits of motors
  limitLower : Inport
  limitUpper : Inport  Port=2
  MATLAB Function : MATLAB Function  TreatAsAtomicUnit=on
  limitVectorZ : Outport
  wires:
  limitLower/1 -> MATLAB Function/1(limLower)
  limitUpper/1 -> MATLAB Function/2(limUpper)
  MATLAB Function/1(limVecZ) -> limitVectorZ/1

== system arducopter/Position Controller/set_pos_target_z_from_climb_rate() ==
  note: input_vel_accel_z()
      | Calculate a jerk limited path from the current position, velocity and acceleration to an input acceleration
  note: set_pos_target_z_from_climb_rate
      | Calculation of target position and desired vel. and accel
  posTarIn : Inport
  climbRateDes : Inport  Port=2
  limitVectorZ : Inport  Port=3
  velMaxUp : Inport  Port=4
  velMaxDn : Inport  Port=5
  accMaxZ : Inport  Port=6
  jerkMaxZ : Inport  Port=7
  posErr : Inport  Port=8
  velErr : Inport  Port=9
  Constant : Constant  Value=0  OutDataTypeStr=single
  Data Store Memory : DataStoreMemory  DataStoreName=velDes  ReadBeforeWriteMsg=warning  WriteAfterWriteMsg=warning  WriteAfterReadMsg=warning  InitialValue=simIn.init.PIDA.velDes  ShowAdditionalParam=off  OutDataTypeStr=single
  Data Store Memory1 : DataStoreMemory  DataStoreName=accDes  ReadBeforeWriteMsg=warning  WriteAfterWriteMsg=warning  WriteAfterReadMsg=warning  InitialValue=simIn.init.PIDA.accDes  ShowAdditionalParam=off  OutDataTypeStr=single
  Data Store Read : DataStoreRead  DataStoreName=velDes  IndexOptions=Index vector (dialog)  Indices=1  OutputSizes=1
  Data Store Read1 : DataStoreRead  DataStoreName=accDes  IndexOptions=Index vector (dialog)  Indices=1  OutputSizes=1
  Data Store Read4 : DataStoreRead  DataStoreName=velDes  IndexOptions=Index vector (dialog)  Indices=1  OutputSizes=1
  Data Store Read5 : DataStoreRead  DataStoreName=accDes  IndexOptions=Index vector (dialog)  Indices=1  OutputSizes=1
  Data Store Write1 : DataStoreWrite  DataStoreName=velDes  IndexOptions=Index vector (dialog)  Indices=1  OutputSizes=1
  Data Store Write2 : DataStoreWrite  DataStoreName=accDes  IndexOptions=Index vector (dialog)  Indices=1  OutputSizes=1
  input_vel_accel_z : Subsystem
  posTar : Outport
  velDes : Outport  Port=2
  accDes : Outport  Port=3
  wires:
  climbRateDes/1 -> input_vel_accel_z/1(velDesTar)
  velMaxUp/1 -> input_vel_accel_z/4(velMaxUp)
  velMaxDn/1 -> input_vel_accel_z/5(velMaxDn)
  accMaxZ/1 -> input_vel_accel_z/6(accMaxZ)
  Constant/1 -> input_vel_accel_z/2(accDesTar)
  jerkMaxZ/1 -> input_vel_accel_z/7(jerkMax)
  limitVectorZ/1 -> input_vel_accel_z/3(limitVectorZ)
  input_vel_accel_z/2(velDes) -> Data Store Write1/1
  input_vel_accel_z/3(accDes) -> Data Store Write2/1
  input_vel_accel_z/1(posTar) -> posTar/1
  Data Store Read4/1 -> velDes/1
  Data Store Read5/1 -> accDes/1
  posTarIn/1 -> input_vel_accel_z/8(posTarIn)
  Data Store Read/1 -> input_vel_accel_z/11(velDesIn)
  Data Store Read1/1 -> input_vel_accel_z/12(accDesIn)
  velErr/1 -> input_vel_accel_z/10(velErr)
  posErr/1 -> input_vel_accel_z/9(posErr)

== system arducopter/Position Controller/zVelCtrlRatio Calculation ==
  note: Update vel_z_control_ratio
      | AC_PosControl.cpp, update_z_controller()
  velErr : Inport
  dnVelMax : Inport  Port=2
  Constant1 : Constant  Value=simIn.param.dt
  Data Store Memory : DataStoreMemory  DataStoreName=vel_z_ctrl_ratio  ReadBeforeWriteMsg=warning  WriteAfterWriteMsg=warning  WriteAfterReadMsg=warning  InitialValue=simIn.param.PSCD.CTRL_RATIO_INIT  ShowAdditionalParam=off  OutDataTypeStr=single
  Data Type Conversion1 : DataTypeConversion  OutDataTypeStr=single
  Update vel_z_ctrl_ratio : MATLAB Function  TreatAsAtomicUnit=on
  zVelCtrlRatio : Outport
  wires:
  Constant1/1 -> Data Type Conversion1/1
  velErr/1 -> Update vel_z_ctrl_ratio/1(velErr)
  dnVelMax/1 -> Update vel_z_ctrl_ratio/2(dnVelMax)
  Data Type Conversion1/1 -> Update vel_z_ctrl_ratio/3(dt)
  Update vel_z_ctrl_ratio/1(zVelCtrlRat) -> zVelCtrlRatio/1

== system arducopter/Rate Controller/Input Handler ==
  note: Actual Values
  note: Desired Values
  note: Use measured desired values for rate controller validation
  note: Use measured actual values for rate controller validation
  inMeas : Inport
  inSim : Inport  Port=2
  Bus Creator : BusCreator  Inputs=6
  Bus Selector : BusSelector  OutputSignals=RATE.rollRateTarMeas,RATE.pitchRateTarMeas,RATE.yawRateTarMeas
  Bus Selector1 : BusSelector  OutputSignals=rollRateTar,pitchRateTar,yawRateTar
  Bus Selector2 : BusSelector  OutputSignals=PIDR.rollRateActMeas,PIDP.pitchRateActMeas,PIDY.yawRateActMeas
  Bus Selector3 : BusSelector  OutputSignals=rollRateAct,pitchRateAct,yawRateAct
  Constant1 : Constant  Value=simIn.param.attCtrlVal
  Constant2 : Constant  Value=simIn.param.attCtrlVal
  Constant3 : Constant  Value=simIn.param.rateCtrlVal
  Constant4 : Constant  Value=simIn.param.rateCtrlVal
  Demux : Demux  Outputs=3
  Demux1 : Demux  Outputs=3
  OR : Logic  Operator=OR  AllPortsSameDT=off  OutDataTypeStr=boolean
  OR1 : Logic  Operator=OR  AllPortsSameDT=off  OutDataTypeStr=boolean
  Switch : Switch  Criteria=u2 > Threshold
  Switch1 : Switch  Criteria=u2 > Threshold
  Vector Concatenate{,1..3} (4 alike) : Concatenate  NumInputs=3
  in : Outport
  wires:
  Bus Creator/1 -> in/1
  inMeas/1 -> Bus Selector2/1, Bus Selector/1
  Bus Selector/1 -> Vector Concatenate/1  "<rollRateTarMeas>"
  Bus Selector/2 -> Vector Concatenate/2  "<pitchRateTarMeas>"
  Bus Selector/3 -> Vector Concatenate/3  "<yawRateTarMeas>"
  inSim/1 -> Bus Selector1/1, Bus Selector3/1
  Bus Selector1/1 -> Vector Concatenate1/1  "<rollRateTar>"
  Bus Selector1/2 -> Vector Concatenate1/2  "<pitchRateTar>"
  Bus Selector1/3 -> Vector Concatenate1/3  "<yawRateTar>"
  Vector Concatenate/1 -> Switch/1
  Vector Concatenate1/1 -> Switch/3
  Bus Selector2/1 -> Vector Concatenate2/1  "<rollRateActMeas>"
  Bus Selector2/2 -> Vector Concatenate2/2  "<pitchRateActMeas>"
  Bus Selector2/3 -> Vector Concatenate2/3  "<yawRateActMeas>"
  Vector Concatenate2/1 -> Switch1/1
  Bus Selector3/1 -> Vector Concatenate3/1  "<rollRateAct>"
  Bus Selector3/2 -> Vector Concatenate3/2  "<pitchRateAct>"
  Bus Selector3/3 -> Vector Concatenate3/3  "<yawRateAct>"
  Vector Concatenate3/1 -> Switch1/3
  Switch/1 -> Demux/1
  Switch1/1 -> Demux1/1
  Demux1/1 -> Bus Creator/4  "rollRateAct"
  Demux1/2 -> Bus Creator/5  "pitchRateAct"
  Demux1/3 -> Bus Creator/6  "yawRateAct"
  Demux/1 -> Bus Creator/1  "rollRateTar"
  Demux/2 -> Bus Creator/2  "pitchRateTar"
  Demux/3 -> Bus Creator/3  "yawRateTar"
  OR/1 -> Switch/2
  Constant4/1 -> OR/1
  Constant1/1 -> OR/2
  Constant2/1 -> OR1/2
  Constant3/1 -> OR1/1
  OR1/1 -> Switch1/2

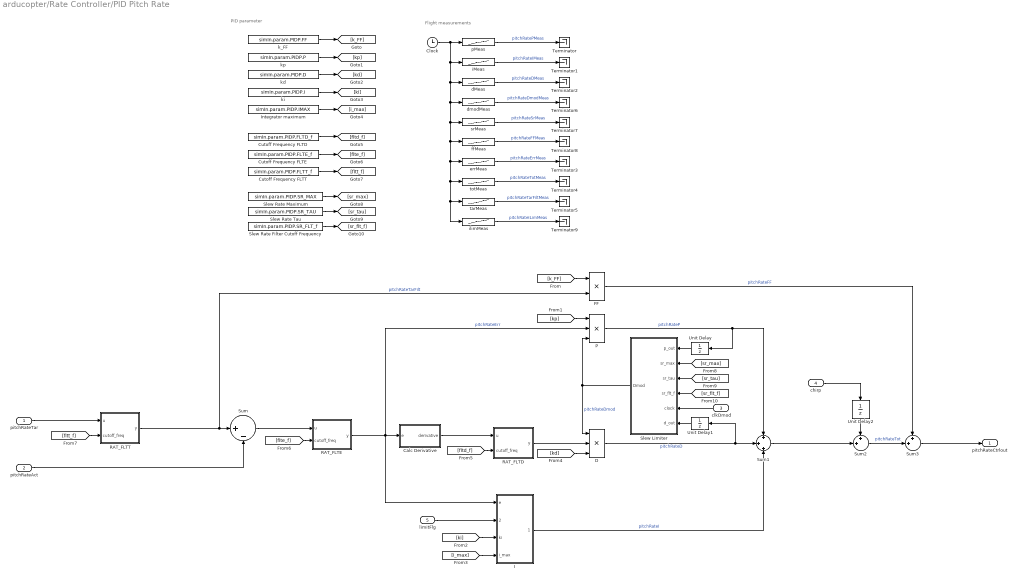
== system arducopter/Rate Controller/PID Pitch Rate ==
  note: PID parameter
  note: Flight measurements
  pitchRateTar : Inport
  pitchRateAct : Inport  Port=2
  clkDmod : Inport  Port=3
  chirp : Inport  Port=4
  limitFlg : Inport  Port=5
  Calc Derivative : Subsystem
  Clock : Clock
  Cutoff Frequency FLTD : Constant  Value=simIn.param.PIDP.FLTD_f
  Cutoff Frequency FLTE : Constant  Value=simIn.param.PIDP.FLTE_f
  Cutoff Frequency FLTT : Constant  Value=simIn.param.PIDP.FLTT_f
  D : Product  Inputs=3
  FF : Product
  I : Subsystem
  Integrator maximum : Constant  Value=simIn.param.PIDP.IMAX
  P : Product  Inputs=3
  RAT_FLTD : Subsystem  TreatAsAtomicUnit=on  SystemSampleTime=simIn.param.dt
  RAT_FLTE : Subsystem  TreatAsAtomicUnit=on  SystemSampleTime=simIn.param.dt
  RAT_FLTT : Subsystem  TreatAsAtomicUnit=on  SystemSampleTime=simIn.param.dt
  Slew Limiter : Subsystem
  Slew Rate Filter Cutoff Frequency : Constant  Value=simIn.param.PIDP.SR_FLT_f
  Slew Rate Maximum : Constant  Value=simIn.param.PIDP.SR_MAX
  Slew Rate Tau : Constant  Value=simIn.param.PIDP.SR_TAU
  Sum : Sum  Inputs=|+-
  Sum1 : Sum  Inputs=+|+|+
  Sum2 : Sum  Inputs=++|
  Sum3 : Sum  Inputs=++|  OutDataTypeStr=single
  Terminator{,1..9} (10 alike) : Terminator
  Unit Delay : UnitDelay  InitialCondition=simIn.init.PIDP.P  SampleTime=-1  HasFrameUpgradeWarning=on
  Unit Delay1 : UnitDelay  InitialCondition=simIn.init.PIDP.D  SampleTime=-1  HasFrameUpgradeWarning=on
  Unit Delay2 : UnitDelay  SampleTime=-1  HasFrameUpgradeWarning=on
  dMeas : Lookup_n-D  NumberOfTableDimensions=1  BreakpointsForDimension1=simIn.signals.PIDP.Time  Table=simIn.signals.PIDP.D  InternalRulePriority=Speed  RndMeth=Simplest  InputSameDT=on
  dmodMeas : Lookup_n-D  NumberOfTableDimensions=1  BreakpointsForDimension1=simIn.signals.PIDP.Time  Table=simIn.signals.PIDP.DMod  InternalRulePriority=Speed  RndMeth=Simplest  InputSameDT=on
  errMeas : Lookup_n-D  NumberOfTableDimensions=1  BreakpointsForDimension1=simIn.signals.PIDP.Time  Table=simIn.signals.PIDP.Err  InternalRulePriority=Speed  RndMeth=Simplest  InputSameDT=on
  ffMeas : Lookup_n-D  NumberOfTableDimensions=1  BreakpointsForDimension1=simIn.signals.PIDP.Time  Table=simIn.signals.PIDP.FF  InternalRulePriority=Speed  RndMeth=Simplest  InputSameDT=on
  iMeas : Lookup_n-D  NumberOfTableDimensions=1  BreakpointsForDimension1=simIn.signals.PIDP.Time  Table=simIn.signals.PIDP.I  InternalRulePriority=Speed  RndMeth=Simplest  InputSameDT=on
  ilimMeas : Lookup_n-D  NumberOfTableDimensions=1  BreakpointsForDimension1=simIn.signals.PIDP.Time  Table=simIn.signals.PIDP.ILimit  InternalRulePriority=Speed  RndMeth=Simplest  InputSameDT=on
  k_FF : Constant  Value=simIn.param.PIDP.FF
  kd : Constant  Value=simIn.param.PIDP.D
  ki : Constant  Value=simIn.param.PIDP.I
  kp : Constant  Value=simIn.param.PIDP.P
  pMeas : Lookup_n-D  NumberOfTableDimensions=1  BreakpointsForDimension1=simIn.signals.PIDP.Time  Table=simIn.signals.PIDP.P  InternalRulePriority=Speed  RndMeth=Simplest  InputSameDT=on
  srMeas : Lookup_n-D  NumberOfTableDimensions=1  BreakpointsForDimension1=simIn.signals.PIDP.Time  Table=simIn.signals.PIDP.SRate  InternalRulePriority=Speed  RndMeth=Simplest  InputSameDT=on
  tarMeas : Lookup_n-D  NumberOfTableDimensions=1  BreakpointsForDimension1=simIn.signals.PIDP.Time  Table=simIn.signals.PIDP.Tar  InternalRulePriority=Speed  RndMeth=Simplest  InputSameDT=on
  totMeas : Lookup_n-D  NumberOfTableDimensions=1  BreakpointsForDimension1=simIn.signals.RATE.Time  Table=simIn.signals.RATE.POut  InternalRulePriority=Speed  RndMeth=Simplest  InputSameDT=on
  pitchRateCtrlout : Outport
  wires:
  [flte_f] -> RAT_FLTE/2(cutoff_freq)
  Cutoff Frequency FLTT/1 -> [fltt_f]
  Cutoff Frequency FLTE/1 -> [flte_f]
  Cutoff Frequency FLTD/1 -> [fltd_f]
  Integrator maximum/1 -> [i_max]
  ki/1 -> [ki]
  kd/1 -> [kd]
  kp/1 -> [kp]
  k_FF/1 -> [k_FF]
  Sum/1 -> RAT_FLTE/1(u)
  pitchRateAct/1 -> Sum/2
  chirp/1 -> Unit Delay2/1
  pitchRateTar/1 -> RAT_FLTT/1(u)
  RAT_FLTT/1(y) -> Sum/1, FF/2  "pitchRateTarFilt"
  Sum2/1 -> Sum3/2  "pitchRateTot"
  I/1(integrator) -> Sum1/3  "pitchRateI"
  D/1 -> Unit Delay1/1, Sum1/2  "pitchRateD"
  Calc Derivative/1(derivative) -> RAT_FLTD/1(u)
  P/1 -> Unit Delay/1, Sum1/1  "pitchRateP"
  limitFlg/1 -> I/2(limit_flg)
  RAT_FLTE/1(y) -> I/1(e), Calc Derivative/1(e), P/2  "pitchRateErr"
  RAT_FLTD/1(y) -> D/2
  pMeas/1 -> Terminator/1  "pitchRatePMeas"
  iMeas/1 -> Terminator1/1  "pitchRateIMeas"
  dMeas/1 -> Terminator2/1  "pitchRateDMeas"
  totMeas/1 -> Terminator4/1  "pitchRateTotMeas"
  tarMeas/1 -> Terminator5/1  "pitchRateTarFiltMeas"
  errMeas/1 -> Terminator3/1  "pitchRateErrMeas"
  Slew Limiter/1(Dmod) -> D/1, P/3  "pitchRateDmod"
  Unit Delay/1 -> Slew Limiter/1(p_out)
  Unit Delay1/1 -> Slew Limiter/6(d_out)
  dmodMeas/1 -> Terminator6/1  "pitchRateDmodMeas"
  srMeas/1 -> Terminator7/1  "pitchRateSrMeas"
  ffMeas/1 -> Terminator8/1  "pitchRateFFMeas"
  Slew Rate Maximum/1 -> [sr_max]
  Slew Rate Tau/1 -> [sr_tau]
  Slew Rate Filter Cutoff Frequency/1 -> [sr_flt_f]
  [sr_max] -> Slew Limiter/2(sr_max)
  [sr_tau] -> Slew Limiter/3(sr_tau)
  [sr_flt_f] -> Slew Limiter/4(sr_flt_f)
  ilimMeas/1 -> Terminator9/1  "pitchRateILimMeas"
  clkDmod/1 -> Slew Limiter/5(clock)
  FF/1 -> Sum3/1  "pitchRateFF"
  Unit Delay2/1 -> Sum2/1
  Clock/1 -> ilimMeas/1, tarMeas/1, totMeas/1, errMeas/1, ffMeas/1, srMeas/1, dmodMeas/1, dMeas/1, iMeas/1, pMeas/1
  Sum1/1 -> Sum2/2
  [i_max] -> I/4(i_max)
  [fltd_f] -> RAT_FLTD/2(cutoff_freq)
  [k_FF] -> FF/1
  [kp] -> P/1
  [kd] -> D/3
  [ki] -> I/3(ki)
  [fltt_f] -> RAT_FLTT/2(cutoff_freq)
  Sum3/1 -> pitchRateCtrlout/1

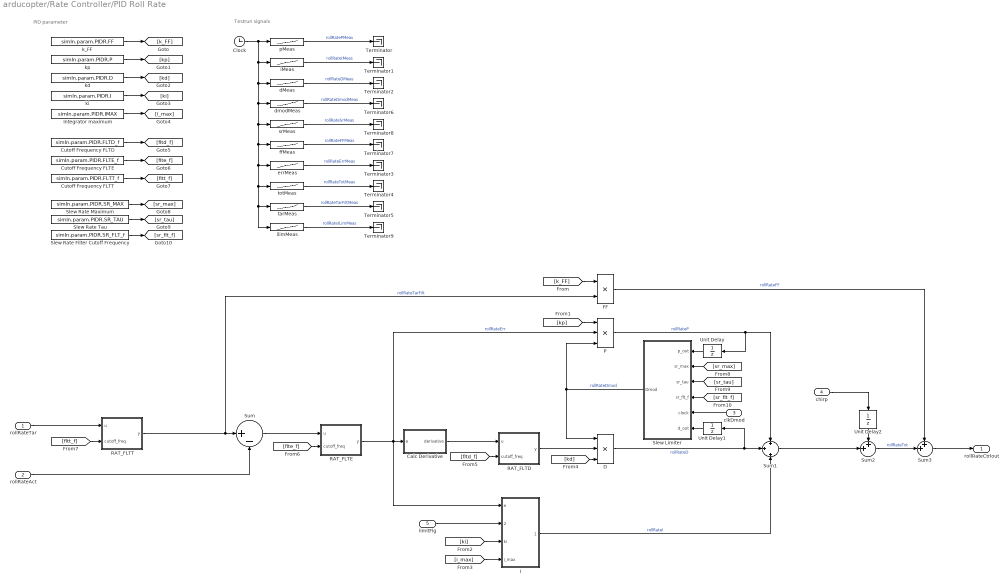
== system arducopter/Rate Controller/PID Roll Rate ==
  note: Testrun signals
  note: PID parameter
  rollRateTar : Inport
  rollRateAct : Inport  Port=2
  clkDmod : Inport  Port=3
  chirp : Inport  Port=4
  limitFlg : Inport  Port=5
  Calc Derivative : Subsystem
  Clock : Clock
  Cutoff Frequency FLTD : Constant  Value=simIn.param.PIDR.FLTD_f
  Cutoff Frequency FLTE : Constant  Value=simIn.param.PIDR.FLTE_f
  Cutoff Frequency FLTT : Constant  Value=simIn.param.PIDR.FLTT_f
  D : Product  Inputs=3
  FF : Product
  I : Subsystem
  Integrator maximum : Constant  Value=simIn.param.PIDR.IMAX
  P : Product  Inputs=3
  RAT_FLTD : Subsystem  TreatAsAtomicUnit=on  SystemSampleTime=simIn.param.dt
  RAT_FLTE : Subsystem  TreatAsAtomicUnit=on  SystemSampleTime=simIn.param.dt
  RAT_FLTT : Subsystem  TreatAsAtomicUnit=on  SystemSampleTime=simIn.param.dt
  Slew Limiter : Subsystem
  Slew Rate Filter Cutoff Frequency : Constant  Value=simIn.param.PIDR.SR_FLT_f
  Slew Rate Maximum : Constant  Value=simIn.param.PIDR.SR_MAX
  Slew Rate Tau : Constant  Value=simIn.param.PIDR.SR_TAU
  Sum : Sum  Inputs=|+-
  Sum1 : Sum  Inputs=+|+|+
  Sum2 : Sum  Inputs=++|
  Sum3 : Sum  Inputs=++|  OutDataTypeStr=single
  Terminator{,1..9} (10 alike) : Terminator
  Unit Delay : UnitDelay  InitialCondition=simIn.init.PIDR.P  SampleTime=-1  HasFrameUpgradeWarning=on
  Unit Delay1 : UnitDelay  InitialCondition=simIn.init.PIDR.D  SampleTime=-1  HasFrameUpgradeWarning=on
  Unit Delay2 : UnitDelay  SampleTime=-1  HasFrameUpgradeWarning=on
  dMeas : Lookup_n-D  NumberOfTableDimensions=1  BreakpointsForDimension1=simIn.signals.PIDR.Time  Table=simIn.signals.PIDR.D  InternalRulePriority=Speed  RndMeth=Simplest  InputSameDT=on
  dmodMeas : Lookup_n-D  NumberOfTableDimensions=1  BreakpointsForDimension1=simIn.signals.PIDR.Time  Table=simIn.signals.PIDR.DMod  InternalRulePriority=Speed  RndMeth=Simplest  InputSameDT=on
  errMeas : Lookup_n-D  NumberOfTableDimensions=1  BreakpointsForDimension1=simIn.signals.PIDR.Time  Table=simIn.signals.PIDR.Err  InternalRulePriority=Speed  RndMeth=Simplest  InputSameDT=on
  ffMeas : Lookup_n-D  NumberOfTableDimensions=1  BreakpointsForDimension1=simIn.signals.PIDR.Time  Table=simIn.signals.PIDR.FF  InternalRulePriority=Speed  RndMeth=Simplest  InputSameDT=on
  iMeas : Lookup_n-D  NumberOfTableDimensions=1  BreakpointsForDimension1=simIn.signals.PIDR.Time  Table=simIn.signals.PIDR.I  InternalRulePriority=Speed  RndMeth=Simplest  InputSameDT=on
  ilimMeas : Lookup_n-D  NumberOfTableDimensions=1  BreakpointsForDimension1=simIn.signals.PIDR.Time  Table=simIn.signals.PIDR.ILimit  InternalRulePriority=Speed  RndMeth=Simplest  InputSameDT=on
  k_FF : Constant  Value=simIn.param.PIDR.FF
  kd : Constant  Value=simIn.param.PIDR.D
  ki : Constant  Value=simIn.param.PIDR.I
  kp : Constant  Value=simIn.param.PIDR.P
  pMeas : Lookup_n-D  NumberOfTableDimensions=1  BreakpointsForDimension1=simIn.signals.PIDR.Time  Table=simIn.signals.PIDR.P  InternalRulePriority=Speed  RndMeth=Simplest  InputSameDT=on
  srMeas : Lookup_n-D  NumberOfTableDimensions=1  BreakpointsForDimension1=simIn.signals.PIDR.Time  Table=simIn.signals.PIDR.SRate  InternalRulePriority=Speed  RndMeth=Simplest  InputSameDT=on
  tarMeas : Lookup_n-D  NumberOfTableDimensions=1  BreakpointsForDimension1=simIn.signals.PIDR.Time  Table=simIn.signals.PIDR.Tar  InternalRulePriority=Speed  RndMeth=Simplest  InputSameDT=on
  totMeas : Lookup_n-D  NumberOfTableDimensions=1  BreakpointsForDimension1=simIn.signals.RATE.Time  Table=simIn.signals.RATE.ROut  InternalRulePriority=Speed  RndMeth=Simplest  InputSameDT=on
  rollRateCtrlout : Outport
  wires:
  RAT_FLTD/1(y) -> D/2
  RAT_FLTE/1(y) -> P/2, Calc Derivative/1(e), I/1(e)  "rollRateErr"
  limitFlg/1 -> I/2(limit_flg)
  P/1 -> Unit Delay/1, Sum1/1  "rollRateP"
  D/1 -> Sum1/2, Unit Delay1/1  "rollRateD"
  I/1(integrator) -> Sum1/3  "rollRateI"
  Sum3/1 -> rollRateCtrlout/1
  RAT_FLTT/1(y) -> FF/2, Sum/1  "rollRateTarFilt"
  rollRateTar/1 -> RAT_FLTT/1(u)
  rollRateAct/1 -> Sum/2
  Sum/1 -> RAT_FLTE/1(u)
  k_FF/1 -> [k_FF]
  kp/1 -> [kp]
  kd/1 -> [kd]
  ki/1 -> [ki]
  Integrator maximum/1 -> [i_max]
  Cutoff Frequency FLTD/1 -> [fltd_f]
  Cutoff Frequency FLTE/1 -> [flte_f]
  Cutoff Frequency FLTT/1 -> [fltt_f]
  [k_FF] -> FF/1
  [kp] -> P/1
  [ki] -> I/3(ki)
  [i_max] -> I/4(i_max)
  [kd] -> D/3
  [fltd_f] -> RAT_FLTD/2(cutoff_freq)
  [flte_f] -> RAT_FLTE/2(cutoff_freq)
  [fltt_f] -> RAT_FLTT/2(cutoff_freq)
  Sum2/1 -> Sum3/2  "rollRateTot"
  pMeas/1 -> Terminator/1  "rollRatePMeas"
  iMeas/1 -> Terminator1/1  "rollRateIMeas"
  errMeas/1 -> Terminator3/1  "rollRateErrMeas"
  dMeas/1 -> Terminator2/1  "rollRateDMeas"
  tarMeas/1 -> Terminator5/1  "rollRateTarFiltMeas"
  totMeas/1 -> Terminator4/1  "rollRateTotMeas"
  Unit Delay/1 -> Slew Limiter/1(p_out)
  Unit Delay1/1 -> Slew Limiter/6(d_out)
  Slew Rate Maximum/1 -> [sr_max]
  [sr_max] -> Slew Limiter/2(sr_max)
  Slew Rate Tau/1 -> [sr_tau]
  Slew Rate Filter Cutoff Frequency/1 -> [sr_flt_f]
  [sr_tau] -> Slew Limiter/3(sr_tau)
  [sr_flt_f] -> Slew Limiter/4(sr_flt_f)
  Slew Limiter/1(Dmod) -> D/1, P/3  "rollRateDmod"
  Sum1/1 -> Sum2/2
  chirp/1 -> Unit Delay2/1
  Unit Delay2/1 -> Sum2/1
  FF/1 -> Sum3/1  "rollRateFF"
  Calc Derivative/1(derivative) -> RAT_FLTD/1(u)
  dmodMeas/1 -> Terminator6/1  "rollRateDmodMeas"
  ffMeas/1 -> Terminator7/1  "rollRateFFMeas"
  srMeas/1 -> Terminator8/1  "rollRateSrMeas"
  clkDmod/1 -> Slew Limiter/5(clock)
  ilimMeas/1 -> Terminator9/1  "rollRateILimMeas"
  Clock/1 -> ilimMeas/1, tarMeas/1, totMeas/1, errMeas/1, ffMeas/1, srMeas/1, dmodMeas/1, dMeas/1, iMeas/1, pMeas/1
